simulink model "calculation"  (R2025b)
settings: Solver=FixedStepDiscrete  StartTime=0  StopTime=T  FixedStep=Ts  RelTol=1e-3
values from neighbouring files (symbols this model uses):
  acceleration = 0.5    [parametrs.m]    (also in solve.m = 2*q*vMean/D)
  bg = 2    [parametrs.m]
  d0 = 0.40    (= 0.4)    [parametrs.m]
  L = delta / 100    (= 0.5)    [parametrs.m]    (also in solve.m = double(L))
  maxRange = FoV * rangeMargin    (= 1.99)    [parametrs.m]
  profileDepth = double(profile.depth_from_side_m(:))    [main.m]
  profileMax = profileX(end)    [main.m]
  profileMin = profileX(1)    [main.m]
  profileX = double(profile.x_m(:))    [main.m]
  speed = 2    [parametrs.m]
  std = 0.003    [parametrs.m]
  Ts = 0.010    (= 0.01)    [parametrs.m]    (also in solve.m = double(Ts))
Description:
  | Сначала main.m: parametrs.m и один MAT-профиль. Затем отдельно Run в Simulink.
settings Model: Creator=Кирилл  LastModifiedBy=Кирилл
settings DataIOCC: SignalLogging=off

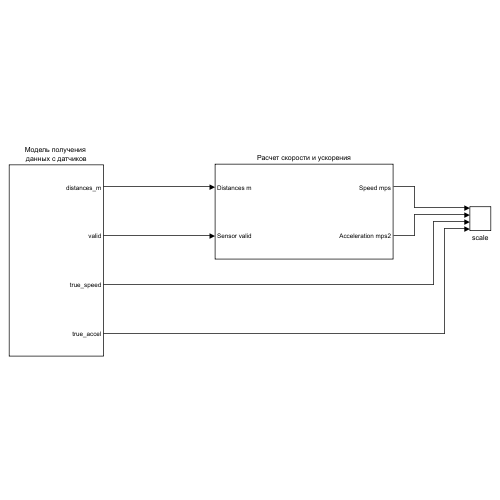
[thumbnail: Simulink's stored preview of the top-level diagram]
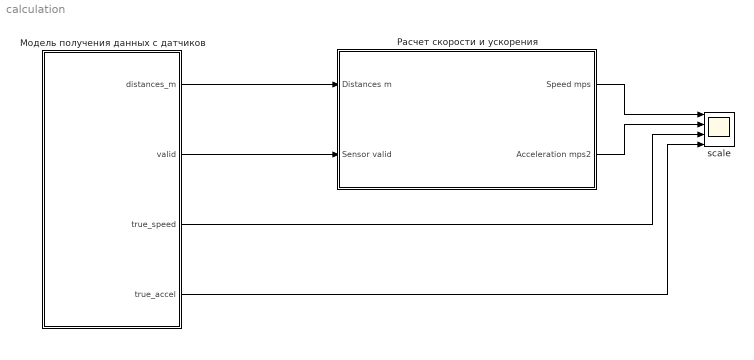
== system calculation ==
  scale : Scope  NumInputPorts=4
      settings: ActiveDisplayYMinimum=-1.5851078626428539  ActiveDisplayYMaximum=10.399078755186656
  Модель получения данных с датчиков : Subsystem
  Расчет скорости и ускорения : Subsystem
  wires:
  Модель получения данных с датчиков/1(distances_m) -> Расчет скорости и ускорения/1(Distances m)
  Модель получения данных с датчиков/2(valid) -> Расчет скорости и ускорения/2(Sensor valid)
  Модель получения данных с датчиков/3(true_speed) -> scale/3
  Модель получения данных с датчиков/4(true_accel) -> scale/4
  Расчет скорости и ускорения/2(Acceleration mps2) -> scale/2
  Расчет скорости и ускорения/1(Speed mps) -> scale/1

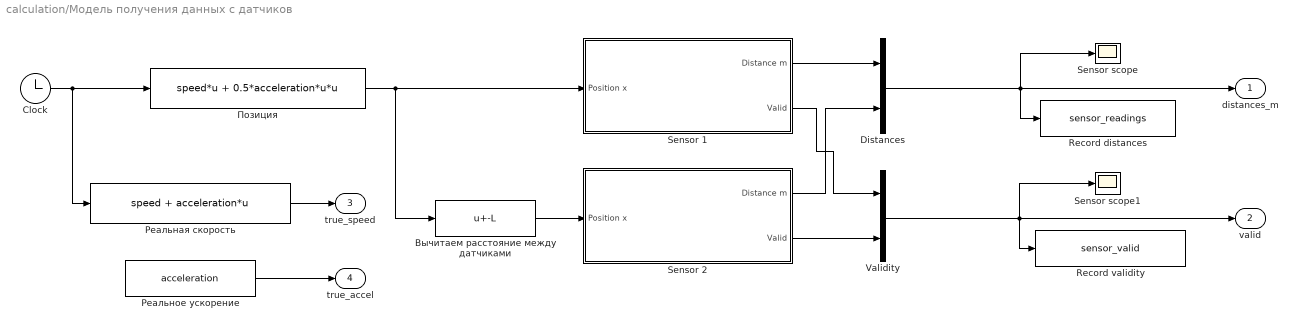
== system calculation/Модель получения данных с датчиков ==
  Clock : Clock
  Distances : Mux  Inputs=2
  Record distances : ToWorkspace  VariableName=sensor_readings  SaveFormat=Timeseries  SampleTime=-1
  Record validity : ToWorkspace  VariableName=sensor_valid  SaveFormat=Timeseries  SampleTime=-1
  Sensor 1 : Subsystem
  Sensor 2 : Subsystem
  Sensor scope : Scope
      settings: ActiveDisplayYMinimum=0.19449298996829029  ActiveDisplayYMaximum=2.2006118900035232
  Sensor scope1 : Scope
      settings: ActiveDisplayYMinimum=-0.12499999999999997  ActiveDisplayYMaximum=1.125
  Validity : Mux  Inputs=2
  "Вычитаем расстояние между датчиками  " : Bias  Bias=-L  SaturateOnIntegerOverflow=off
  "Позиция " : Fcn  Expr=speed*u + 0.5*acceleration*u*u
  Реальная скорость : Fcn  Expr=speed + acceleration*u
  Реальное ускорение : Constant  Value=acceleration  SampleTime=Ts
  distances_m : Outport
  valid : Outport  Port=2
  true_speed : Outport  Port=3
  true_accel : Outport  Port=4
  wires:
  Sensor 1/2(Valid) -> Validity/1
  Distances/1 -> distances_m/1, Sensor scope/1, Record distances/1
  "Позиция "/1 -> "Вычитаем расстояние между датчиками  "/1, Sensor 1/1(Position x)
  Sensor 1/1(Distance m) -> Distances/1
  Clock/1 -> "Позиция "/1, Реальная скорость/1
  Sensor 2/2(Valid) -> Validity/2
  "Вычитаем расстояние между датчиками  "/1 -> Sensor 2/1(Position x)
  Реальное ускорение/1 -> true_accel/1
  Validity/1 -> valid/1, Sensor scope1/1, Record validity/1
  Sensor 2/1(Distance m) -> Distances/2
  Реальная скорость/1 -> true_speed/1

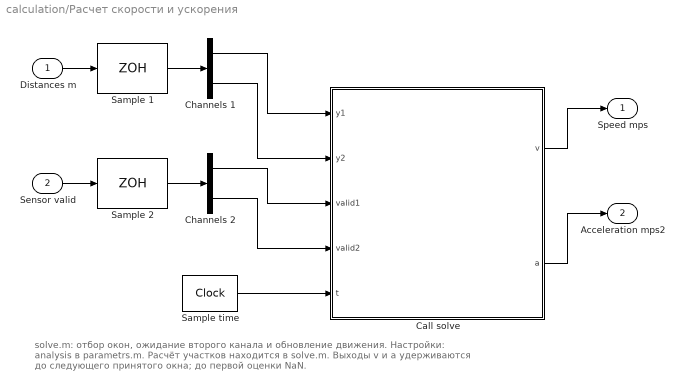
== system calculation/Расчет скорости и ускорения ==
  note: solve.m: отбор окон, ожидание второго канала и обновление движения.
      | Настройки: analysis в parametrs.m. Расчёт участков находится в solve.m.
      | Выходы v и a удерживаются до следующего принятого окна; до первой оценки NaN.
  Distances m : Inport
  Sensor valid : Inport  Port=2
  Call solve : MATLAB Function  TreatAsAtomicUnit=on
  Channels 1 : Demux  Outputs=2
  Channels 2 : Demux  Outputs=2
  Sample 1 : ZeroOrderHold  SampleTime=Ts
  Sample 2 : ZeroOrderHold  SampleTime=Ts
  Sample time : DigitalClock  SampleTime=Ts
  Speed mps : Outport
  Acceleration mps2 : Outport  Port=2
  wires:
  Distances m/1 -> Sample 1/1
  Sensor valid/1 -> Sample 2/1
  Sample 1/1 -> Channels 1/1
  Sample 2/1 -> Channels 2/1
  Channels 1/1 -> Call solve/1(y1)
  Channels 1/2 -> Call solve/2(y2)
  Channels 2/1 -> Call solve/3(valid1)
  Channels 2/2 -> Call solve/4(valid2)
  Sample time/1 -> Call solve/5(t)
  Call solve/1(v) -> Speed mps/1
  Call solve/2(a) -> Acceleration mps2/1

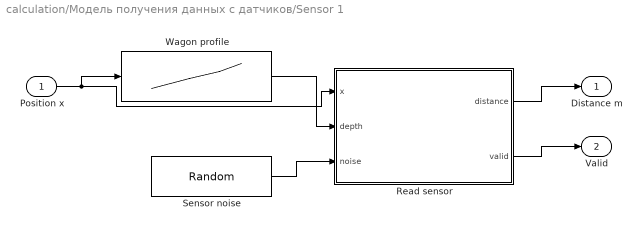
== system calculation/Модель получения данных с датчиков/Sensor 1 ==
  Position x : Inport
  Read sensor : MATLAB Function  TreatAsAtomicUnit=on
  Sensor noise : RandomNumber  Variance=std^2  Seed=11  SampleTime=Ts
  Wagon profile : Lookup_n-D  NumberOfTableDimensions=1  BreakpointsForDimension1=profileX  Table=profileDepth  ExtrapMethod=Clip  InternalRulePriority=Speed  RndMeth=Simplest
  Distance m : Outport
  Valid : Outport  Port=2
  wires:
  Position x/1 -> Wagon profile/1, Read sensor/1(x)
  Wagon profile/1 -> Read sensor/2(depth)
  Sensor noise/1 -> Read sensor/3(noise)
  Read sensor/1(distance) -> Distance m/1
  Read sensor/2(valid) -> Valid/1

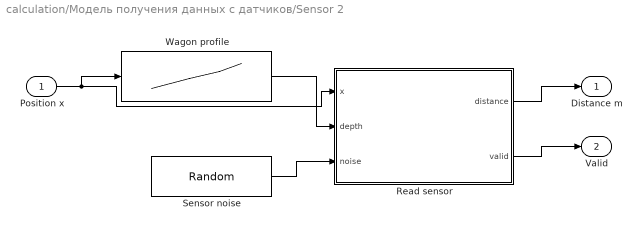
== system calculation/Модель получения данных с датчиков/Sensor 2 ==
  Position x : Inport
  Read sensor : MATLAB Function  TreatAsAtomicUnit=on
  Sensor noise : RandomNumber  Variance=std^2  Seed=29  SampleTime=Ts
  Wagon profile : Lookup_n-D  NumberOfTableDimensions=1  BreakpointsForDimension1=profileX  Table=profileDepth  ExtrapMethod=Clip  InternalRulePriority=Speed  RndMeth=Simplest
  Distance m : Outport
  Valid : Outport  Port=2
  wires:
  Position x/1 -> Wagon profile/1, Read sensor/1(x)
  Wagon profile/1 -> Read sensor/2(depth)
  Sensor noise/1 -> Read sensor/3(noise)
  Read sensor/1(distance) -> Distance m/1
  Read sensor/2(valid) -> Valid/1

== matlab function calculation/Модель получения данных с датчиков/Sensor 2/Read sensor ==
  data: x input; distance output; depth input; noise input; valid output; d0 parameter; profileMin parameter; profileMax parameter; maxRange parameter; bg parameter
function [distance, valid] = read_sensor(x, depth, noise, d0, profileMin, profileMax, maxRange, bg)
%#codegen
raw = d0 + depth + noise;
valid = x >= profileMin && x <= profileMax && raw > 0 && raw <= maxRange;
if valid
    distance = raw;
else
    distance = bg;
end
end

== matlab function calculation/Модель получения данных с датчиков/Sensor 1/Read sensor ==
  data: x input; distance output; depth input; noise input; valid output; d0 parameter; profileMin parameter; profileMax parameter; maxRange parameter; bg parameter
function [distance, valid] = read_sensor(x, depth, noise, d0, profileMin, profileMax, maxRange, bg)
%#codegen
raw = d0 + depth + noise;
valid = x >= profileMin && x <= profileMax && raw > 0 && raw <= maxRange;
if valid
    distance = raw;
else
    distance = bg;
end
end

== matlab function calculation/Расчет скорости и ускорения/Call solve ==
  data: y1 input; v output; y2 input; valid1 input; valid2 input; t input; a output; analysis parameter
function [v,a] = estimate(y1,y2,valid1,valid2,t,analysis)
%#codegen
coder.extrinsic('solve');
v=NaN; a=NaN;
[v,a]=solve(y1,y2,valid1,valid2,t,analysis);
end
